simulink model "SecondOrderSystem"  (R2024b)
settings: Solver=VariableStepAuto  StartTime=0.0  StopTime=10.0  RelTol=1e-3
settings Model: Creator=33242  LastModifiedBy=33242

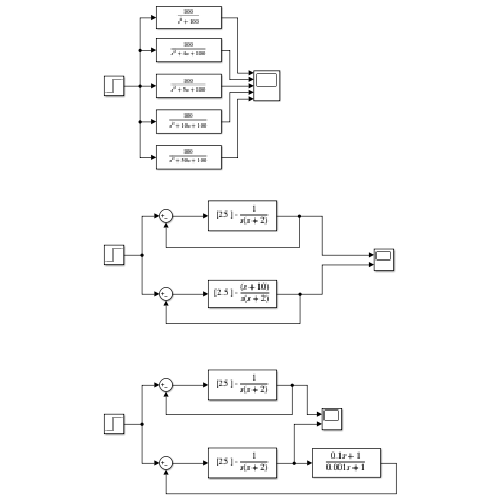
[thumbnail: Simulink's stored preview of the top-level diagram]
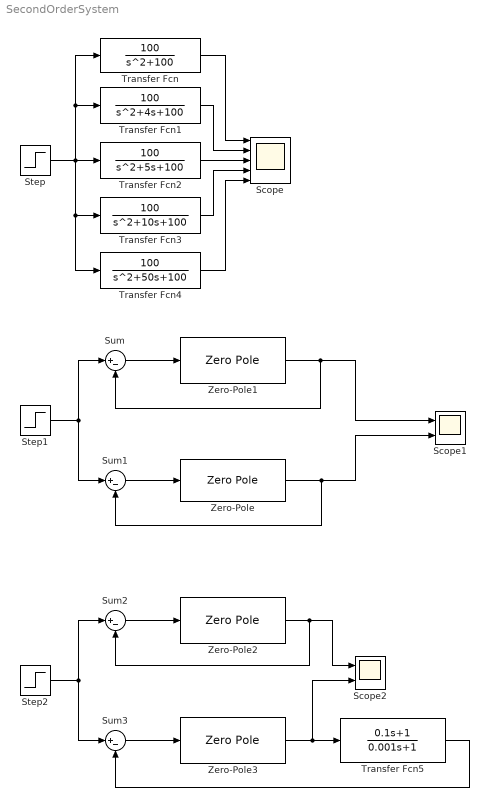
== system SecondOrderSystem ==
  Scope : Scope  NumInputPorts=5
  Scope1 : Scope  NumInputPorts=2
  Scope2 : Scope  NumInputPorts=2
  Step : Step  SampleTime=0
  Step1 : Step  SampleTime=0
  Step2 : Step  SampleTime=0
  Sum{,1..3} (4 alike) : Sum  Inputs=|+-
  Transfer Fcn : TransferFcn  Numerator=[100]  Denominator=[1 0 100]
  Transfer Fcn1 : TransferFcn  Numerator=[100]  Denominator=[1 4 100]
  Transfer Fcn2 : TransferFcn  Numerator=[100]  Denominator=[1 5 100]
  Transfer Fcn3 : TransferFcn  Numerator=[100]  Denominator=[1 10 100]
  Transfer Fcn4 : TransferFcn  Numerator=[100]  Denominator=[1 50 100]
  Transfer Fcn5 : TransferFcn  Numerator=[0.1 1]  Denominator=[0.001 1]
  Zero-Pole : ZeroPole  Zeros=[-10]  Poles=[0 -2]  Gain=[2.5]
  Zero-Pole1 : ZeroPole  Zeros=[]  Poles=[0 -2]  Gain=[25]
  Zero-Pole2 : ZeroPole  Zeros=[]  Poles=[0 -2]  Gain=[25]
  Zero-Pole3 : ZeroPole  Zeros=[]  Poles=[0 -2]  Gain=[25]
  wires:
  Step/1 -> Transfer Fcn/1, Transfer Fcn1/1, Transfer Fcn4/1, Transfer Fcn3/1, Transfer Fcn2/1
  Transfer Fcn/1 -> Scope/1
  Transfer Fcn1/1 -> Scope/2
  Transfer Fcn2/1 -> Scope/3
  Transfer Fcn4/1 -> Scope/5
  Transfer Fcn3/1 -> Scope/4
  Step1/1 -> Sum1/1, Sum/1
  Sum/1 -> Zero-Pole1/1
  Sum1/1 -> Zero-Pole/1
  Zero-Pole1/1 -> Scope1/1, Sum/2
  Zero-Pole/1 -> Scope1/2, Sum1/2
  Step2/1 -> Sum2/1, Sum3/1
  Sum2/1 -> Zero-Pole2/1
  Sum3/1 -> Zero-Pole3/1
  Zero-Pole3/1 -> Scope2/2, Transfer Fcn5/1
  Zero-Pole2/1 -> Scope2/1, Sum2/2
  Transfer Fcn5/1 -> Sum3/2
